simulink model "Impl_Sprayer"  (R2026b)
settings: Solver=VariableStepAuto
undefined symbols (not defined in the file or in its folder): P, Ts
libraries: fl_lib x8, nesl_utility x7, simulink x5, ee_lib x4
settings Model: Creator=aomar  LastModifiedBy=aomar

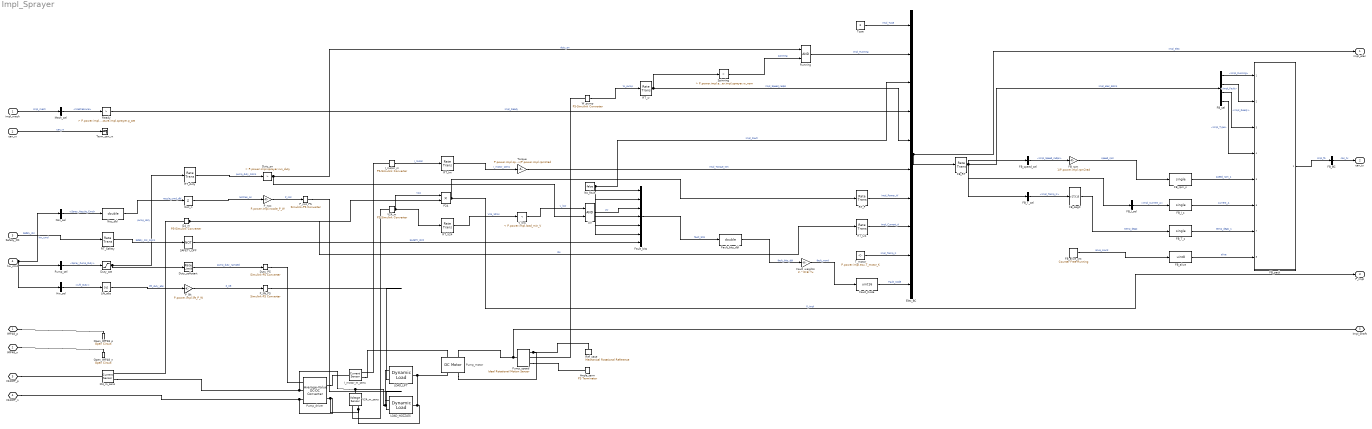
== system Impl_Sprayer ==
  impl_mech : Inport  OutDataTypeStr=Bus: Bus_ImplMechState  SampleTime=Ts.ctrl
  can_rx : Inport  Port=2  OutDataTypeStr=Bus: Bus_Can1_McuSlow  SampleTime=Ts.can_slow
  Safety_OK : Inport  Port=3  OutDataTypeStr=boolean  SampleTime=Ts.safety
  hw_cmd : Inport  Port=4  OutDataTypeStr=Bus: Bus_PowerHwCmd  SampleTime=Ts.base
  Angle_term : fl_lib/Physical Signals/Sinks/PS Terminator
  Duty_PS : nesl_utility/Simulink-PS Converter  PhysicalDomain=network_engine_domain  SubClassName=ps_input  LeftPortType=input  RightPortType=output  PseudoPeriodic=off  Frequencies=[]  NoiseDistribution=none  NoiseParameters=[]  Unit=1  AffineConversion=off  FilteringAndDerivatives=zero  SimscapeFilterOrder=1  InputFilterTimeConstant=0.001  UdotUserProvided=0
  Duty_on : simulink/Logic and Bit Operations/Compare To Constant  relop=>  const=P.power.impl.sprayer.run_duty  OutDataTypeStr=boolean
  Duty_sat : Saturate  UpperLimit=1  LowerLimit=0
  Duty_softstart : RateLimiter  RisingSlewLimit=P.power.impl.sprayer.duty_slew  FallingSlewLimit=-1e3  SampleTimeMode=inherited
  Elec_BC : BusCreator  Inputs=10  OutDataTypeStr=Bus: Bus_ImplElecState  NonVirtualBus=on
      settings: InheritFromInputs=off
  FB_BC : BusCreator  Inputs=1  OutDataTypeStr=Bus: Bus_Can1_Impl  NonVirtualBus=on
      settings: InheritFromInputs=off
  FB_I_s : DataTypeConversion  OutDataTypeStr=single  SaturateOnIntegerOverflow=off  RndMeth=Floor
  FB_I_sel : BusSelector  OutputSignals=Impl_Current_A
  FB_RT : RateTransition  OutPortSampleTime=Ts.can_slow
  FB_T_s : DataTypeConversion  OutDataTypeStr=single  SaturateOnIntegerOverflow=off  RndMeth=Floor
  FB_T_sel : BusSelector  OutputSignals=Impl_Temp_K
  FB_alive : DataTypeConversion  OutDataTypeStr=uint8  SaturateOnIntegerOverflow=off  RndMeth=Floor
  FB_alive_cnt : simulink/Sources/Counter Free-Running  NumBits=8  tsamp=Ts.can_slow
  FB_degC : Bias  Bias=-273.15  SaturateOnIntegerOverflow=off
  FB_pack : Subsystem  ReferencedSubsystem=implfb_can_pack
  FB_rpm : Gain  Gain=1/P.power.impl.rpm2rad
  FB_rpm_s : DataTypeConversion  OutDataTypeStr=single  SaturateOnIntegerOverflow=off  RndMeth=Floor
  FB_sel : BusSelector  OutputSignals=Impl_Running,Impl_Fault,Impl_Ready,Impl_Type
  FB_speed_sel : BusSelector  OutputSignals=Impl_Speed_radps
  Fault_Code : DataTypeConversion  OutDataTypeStr=uint16  RndMeth=Nearest
  Fault_bits : Mux  Inputs=7
  Fault_bits_dbl : DataTypeConversion  OutDataTypeStr=double  SaturateOnIntegerOverflow=off  RndMeth=Floor
  Fault_weights : Gain  Gain=2.^(0:6)  Multiplication=Matrix(K*u)
  Hw_sel : BusSelector  OutputSignals=Lift_Duty
  I24_m : nesl_utility/PS-Simulink Converter  PhysicalDomain=network_engine_domain  SubClassName=ps_output  LeftPortType=input  RightPortType=output  PseudoPeriodic=off  Frequencies=[]  VectorFormat=inherit  Unit=A  AffineConversion=off
  I24_m_sens : fl_lib/Electrical/Electrical Sensors/Current Sensor
  I_motor_m : nesl_utility/PS-Simulink Converter  PhysicalDomain=network_engine_domain  SubClassName=ps_output  LeftPortType=input  RightPortType=output  PseudoPeriodic=off  Frequencies=[]  VectorFormat=inherit  Unit=A  AffineConversion=off
  I_motor_m_sens : fl_lib/Electrical/Electrical Sensors/Current Sensor
  LOAD_LIFT : ee_lib/Passive/Dynamic Load  load_type=ee.enum.dc_ac.dc  min_supply_voltage=P.power.impl.load_min_V V  pow_min=P.power.lv.load.pow_min W  G_reverse=P.power.lv.load.G_reverse S  deltaV=P.power.lv.load.deltaV V  f0=60 Hz  Vrms_min=200 V  tau=0.01 s  Vrms_ini=300 V  Vang_ini=0 deg
  LOAD_NOZZLES : ee_lib/Passive/Dynamic Load  load_type=ee.enum.dc_ac.dc  min_supply_voltage=P.power.impl.load_min_V V  pow_min=P.power.lv.load.pow_min W  G_reverse=P.power.lv.load.G_reverse S  deltaV=P.power.lv.load.deltaV V  f0=60 Hz  Vrms_min=200 V  tau=0.01 s  Vrms_ini=300 V  Vang_ini=0 deg
  Lift_abs : Abs  SaturateOnIntegerOverflow=off
  Mech_sel : BusSelector  OutputSignals=linePressure
  No_fault : Constant  Value=false  OutDataTypeStr=boolean  SampleTime=Ts.impl_ctrl
  Noz_dbl : DataTypeConversion  OutDataTypeStr=double  SaturateOnIntegerOverflow=off  RndMeth=Floor
  Noz_n : Sum  Inputs=+
  Noz_sel : BusSelector  OutputSignals=Spray_Nozzle_Cmd
  Open_IMP48_n : fl_lib/Electrical/Electrical Elements/Open Circuit  v_specify=off  v_priority=None  v=0 V  v_nominal_specify=off  v_nominal_value=1  v_nominal_unit=V
      settings: LibrarySourceBlock=|
      | ee_lib/Connectors &
      | References/Open Circuit
  Open_IMP48_p : fl_lib/Electrical/Electrical Elements/Open Circuit  v_specify=off  v_priority=None  v=0 V  v_nominal_specify=off  v_nominal_value=1  v_nominal_unit=V
      settings: LibrarySourceBlock=|
      | ee_lib/Connectors &
      | References/Open Circuit
  P24 : Product
  P_lift : Gain  Gain=P.power.impl.lift_P_W
  P_lift_PS : nesl_utility/Simulink-PS Converter  PhysicalDomain=network_engine_domain  SubClassName=ps_input  LeftPortType=input  RightPortType=output  PseudoPeriodic=off  Frequencies=[]  NoiseDistribution=none  NoiseParameters=[]  Unit=W  AffineConversion=off  FilteringAndDerivatives=zero  SimscapeFilterOrder=1  InputFilterTimeConstant=0.001  UdotUserProvided=0
  P_noz : Gain  Gain=P.power.impl.nozzle_P_W
  P_noz_PS : nesl_utility/Simulink-PS Converter  PhysicalDomain=network_engine_domain  SubClassName=ps_input  LeftPortType=input  RightPortType=output  PseudoPeriodic=off  Frequencies=[]  NoiseDistribution=none  NoiseParameters=[]  Unit=W  AffineConversion=off  FilteringAndDerivatives=zero  SimscapeFilterOrder=1  InputFilterTimeConstant=0.001  UdotUserProvided=0
  Pump_driver : ee_lib/Semiconductors & Converters/Converters/Average-Value DC-DC Converter  implementation_option=ee.enum.converters.implementation.behavioral  converter_type=ee.enum.converters.dcdctype.buck  control_option=ee.enum.converters.controlinput.dutycycle  efficiency_option=ee.enum.converters.efficiency.constant  efficiency_fixed=P.power.impl.sprayer.buck_eff  i_vec=[0, 2, 5] A  efficiency_vec=[90, 95, 98]  Lf=1e-6 H  Rl=0 Ohm  Cf=1e-7 F  Rc=1e-6 Ohm  iL_specify=off  iL_priority=High  iL=0 A  iL_nominal_specify=off  iL_nominal_value=1  iL_nominal_unit=A  vc_specify=off  vc_priority=High  vc=0 V  vc_nominal_specify=off  vc_nominal_value=1  vc_nominal_unit=V
  Pump_motor : ee_lib/Electromechanical/Brushed Motors/DC Motor  field_option=ee.enum.field_option.pm  Rf=100 Ohm  Lf=1 H  Laf=0.15 H  If0=0 A  parameterization=ee.enum.dcparam_option.circuit_param  Ra=P.power.impl.sprayer.Ra Ohm  La=P.power.impl.sprayer.La H  emf_or_torque=ee.enum.emf_or_torque.kv  Kv=P.power.impl.sprayer.Kv V/rpm  Ki=6.876e-4 N*m/A  T_stall=0.24e-3 N*m  w_max=19100 rpm  w_rated=15000 rpm  P_rated=0.08 W  V_rated=1.5 V  lam_param=ee.enum.lam_param.damping  i_noload=0 A  V_i_noload=1.5 V  J=P.power.impl.sprayer.J kg*m^2  lam=P.power.impl.sprayer.lam N*m*s/rad  speed0=0 rpm  alpha=3.93e-3 1/K  Tmeas=25 degC  thermal_mass=100 J/K  initial_temperature=25 degC
  Pump_sel : BusSelector  OutputSignals=Spray_Pump_Duty
  Pump_speed : fl_lib/Mechanical/Mechanical Sensors/Ideal Rotational Motion Sensor  reference=foundation.enum.MeasurementReference.difference  acceleration_port=false  velocity_port=true  position_port=true  wrap_angle=false  offset=0 rad
  RT_I24 : RateTransition  OutPortSampleTime=Ts.impl_ctrl
  RT_Im : RateTransition  OutPortSampleTime=Ts.impl_ctrl
  RT_P : RateTransition  OutPortSampleTime=Ts.impl_ctrl
  RT_Safety : RateTransition  OutPortSampleTime=Ts.impl_ctrl
  RT_V24 : RateTransition  OutPortSampleTime=Ts.impl_ctrl
  RT_duty : RateTransition  OutPortSampleTime=Ts.impl_ctrl
  RT_w : RateTransition  OutPortSampleTime=Ts.impl_ctrl
  Ready : simulink/Logic and Bit Operations/Compare To Constant  relop=>  const=P.power.impl.sprayer.p_ready_frac*P.structure.impl.sprayer.p_set  OutDataTypeStr=boolean
  Ref_case : fl_lib/Mechanical/Rotational Elements/Mechanical Rotational Reference
  Running : Logic  AllPortsSameDT=off  OutDataTypeStr=boolean
  SAFETY_OFF : Logic  Operator=NOT  AllPortsSameDT=off  OutDataTypeStr=boolean
  Spinning : simulink/Logic and Bit Operations/Compare To Constant  relop=>  const=P.power.impl.ecu.run_frac*P.power.impl.sprayer.w_nom  OutDataTypeStr=boolean
  T_motor : Constant  Value=P.power.impl.ecu.T_motor_K  SampleTime=Ts.impl_ctrl
  Term_can_rx : Terminator
  Torque : Gain  Gain=P.power.impl.sprayer.Kv/P.power.impl.rpm2rad
  Type : Constant  Value=3  OutDataTypeStr=uint8  SampleTime=Ts.impl_ctrl
  UV : Logic  AllPortsSameDT=off  OutDataTypeStr=boolean
  V24_m : nesl_utility/PS-Simulink Converter  PhysicalDomain=network_engine_domain  SubClassName=ps_output  LeftPortType=input  RightPortType=output  PseudoPeriodic=off  Frequencies=[]  VectorFormat=inherit  Unit=V  AffineConversion=off
  V24_m_sens : fl_lib/Electrical/Electrical Sensors/Voltage Sensor
  V_low : simulink/Logic and Bit Operations/Compare To Constant  relop=<  const=P.power.impl.load_min_V  OutDataTypeStr=boolean
  W_pump : nesl_utility/PS-Simulink Converter  PhysicalDomain=network_engine_domain  SubClassName=ps_output  LeftPortType=input  RightPortType=output  PseudoPeriodic=off  Frequencies=[]  VectorFormat=inherit  Unit=rad/s  AffineConversion=off
  IMP48_p : PMIOPort  Side=Left  ConnectionType=Connection: foundation.electrical.electrical
  IMP48_n : PMIOPort  Port=2  Side=Left  ConnectionType=Connection: foundation.electrical.electrical
  V24IMP_p : PMIOPort  Port=3  Side=Left  ConnectionType=Connection: foundation.electrical.electrical
  V24IMP_n : PMIOPort  Port=4  Side=Left  ConnectionType=Connection: foundation.electrical.electrical
  Impl_Shaft : PMIOPort  Port=5  Side=Right  ConnectionType=Connection: foundation.mechanical.rotational.rotational
  impl_elec : Outport  OutDataTypeStr=Bus: Bus_ImplElecState
  can_tx : Outport  Port=2  OutDataTypeStr=Bus: Bus_Can1_Impl
  P_impl : Outport  Port=3  OutDataTypeStr=double
  wires:
  impl_mech/1 -> Mech_sel/1  "impl_mech"
  can_rx/1 -> Term_can_rx/1  "can_rx"
  Safety_OK/1 -> RT_Safety/1  "Safety_OK"
  hw_cmd/1 -> Noz_sel/1, Hw_sel/1, Pump_sel/1  "hw_cmd"
  Mech_sel/1 -> Ready/1  "<linePressure>"
  Noz_sel/1 -> Noz_dbl/1  "<Spray_Nozzle_Cmd>"
  Pump_sel/1 -> Duty_sat/1  "<Spray_Pump_Duty>"
  Hw_sel/1 -> Lift_abs/1  "<Lift_Duty>"
  Ready/1 -> Elec_BC/4  "Impl_Ready"
  Duty_sat/1 -> RT_duty/1, Duty_softstart/1  "pump_duty"
  Lift_abs/1 -> P_lift/1  "lift_duty_abs"
  RT_Safety/1 -> SAFETY_OFF/1  "Safety_OK_10ms"
  Noz_dbl/1 -> Noz_n/1  "nozzle_cmd_dbl"
  I24_m/1 -> P24/2, RT_I24/1  "I24"
  Noz_n/1 -> P_noz/1  "nozzles_on"
  SAFETY_OFF/1 -> Fault_bits/7  "SAFETY_OFF"
  Duty_softstart/1 -> Duty_PS/1  "pump_duty_ramped"
  P_lift/1 -> P_lift_PS/1  "P_lift"
  RT_duty/1 -> Duty_on/1  "pump_duty_10ms"
  Duty_on/1 -> Running/1, UV/2  "duty_on"
  P_noz/1 -> P_noz_PS/1  "P_noz"
  I_motor_m/1 -> RT_Im/1  "I_motor"
  V24_m/1 -> RT_V24/1, P24/1  "V24"
  P24/1 -> P_impl/1, RT_P/1  "P_impl"
  RT_Im/1 -> Torque/1  "I_motor_10ms"
  RT_V24/1 -> V_low/1  "V24_10ms"
  Torque/1 -> Elec_BC/6  "Impl_Torque_Nm"
  V_low/1 -> UV/1  "v_low"
  W_pump/1 -> RT_w/1  "W_pump"
  No_fault/1 -> Elec_BC/3, Fault_bits/6, Fault_bits/5, Fault_bits/4, Fault_bits/2, Fault_bits/1  "Impl_Fault"
  UV/1 -> Fault_bits/3  "UV"
  Fault_bits/1 -> Fault_bits_dbl/1  "fault_bits"
  RT_w/1 -> Elec_BC/5, Spinning/1  "Impl_Speed_radps"
  Spinning/1 -> Running/2  "spinning"
  Fault_bits_dbl/1 -> Fault_weights/1  "fault_bits_dbl"
  Running/1 -> Elec_BC/2  "Impl_Running"
  Fault_weights/1 -> Fault_Code/1  "fault_word"
  Type/1 -> Elec_BC/1  "Impl_Type"
  T_motor/1 -> Elec_BC/9  "Impl_Temp_K"
  RT_P/1 -> Elec_BC/7  "Impl_Power_W"
  RT_I24/1 -> Elec_BC/8  "Impl_Current_A"
  Fault_Code/1 -> Elec_BC/10  "Fault_Code"
  Elec_BC/1 -> impl_elec/1, FB_RT/1  "impl_elec"
  FB_RT/1 -> FB_sel/1, FB_I_sel/1, FB_T_sel/1, FB_speed_sel/1  "impl_elec_50ms"
  FB_speed_sel/1 -> FB_rpm/1  "<Impl_Speed_radps>"
  FB_T_sel/1 -> FB_degC/1  "<Impl_Temp_K>"
  FB_rpm/1 -> FB_rpm_s/1  "speed_rpm"
  FB_alive_cnt/1 -> FB_alive/1  "alive_count"
  FB_degC/1 -> FB_T_s/1  "temp_degC"
  FB_I_sel/1 -> FB_I_s/1  "<Impl_Current_A>"
  FB_rpm_s/1 -> FB_pack/5  "speed_rpm_s"
  FB_I_s/1 -> FB_pack/6  "current_A"
  FB_T_s/1 -> FB_pack/7  "temp_degC_s"
  FB_alive/1 -> FB_pack/8  "alive"
  FB_sel/1 -> FB_pack/1  "<Impl_Running>"
  FB_sel/2 -> FB_pack/2  "<Impl_Fault>"
  FB_sel/3 -> FB_pack/3  "<Impl_Ready>"
  FB_sel/4 -> FB_pack/4  "<Impl_Type>"
  FB_pack/1 -> FB_BC/1  "impl_fb"
  FB_BC/1 -> can_tx/1  "can_tx"
  connections:
  Pump_speed/RConn3 -- Angle_term/LConn1
  Duty_PS/RConn1 -- Pump_driver/LConn1
  I24_m/LConn1 -- I24_m_sens/RConn1
  V24IMP_p/RConn1 -- I24_m_sens/LConn1
  Pump_driver/LConn2 -- I24_m_sens/RConn2 -- V24_m_sens/LConn1 -- LOAD_NOZZLES/LConn1 -- LOAD_LIFT/LConn1
  IMP48_n/RConn1 -- Open_IMP48_n/LConn1
  IMP48_p/RConn1 -- Open_IMP48_p/LConn1
  I_motor_m/LConn1 -- I_motor_m_sens/RConn1
  Pump_driver/RConn1 -- I_motor_m_sens/LConn1
  I_motor_m_sens/RConn2 -- Pump_motor/LConn1
  Pump_speed/LConn1 -- Pump_motor/LConn2 -- Impl_Shaft/RConn1
  P_lift_PS/RConn1 -- LOAD_LIFT/LConn2
  Pump_driver/LConn3 -- V24IMP_n/RConn1 -- Pump_driver/RConn2 -- V24_m_sens/RConn2 -- LOAD_NOZZLES/RConn1 -- LOAD_LIFT/RConn1 -- Pump_motor/RConn1
  P_noz_PS/RConn1 -- LOAD_NOZZLES/LConn2
  Pump_speed/RConn1 -- Pump_motor/RConn2 -- Ref_case/LConn1
  W_pump/LConn1 -- Pump_speed/RConn2
  V24_m/LConn1 -- V24_m_sens/RConn1
